simulink model "simscapePMSM"  (R2023b)
settings: Solver=VariableStepAuto  StartTime=0.0  StopTime=0.6  MaxStep=1e-4  RelTol=1e-3
undefined symbols (not defined in the file): Ld, Lq, Phif
libraries: slpidlib x2, spsDCVoltageSourceLib x1, mcbcontrolslib x1, spsPWMGenerator2LevelLib x1, eeTransforms x1, spsPermanentMagnetSynchronousMachineLib x1, spsUniversalBridgeLib x1, sps_lib x1
settings Model: Creator=HP  LastModifiedBy=HP
settings SolverCC: ZeroCrossAlgorithm=Adaptive
settings DebuggingCC: IgnoredZcDiagnostic=none

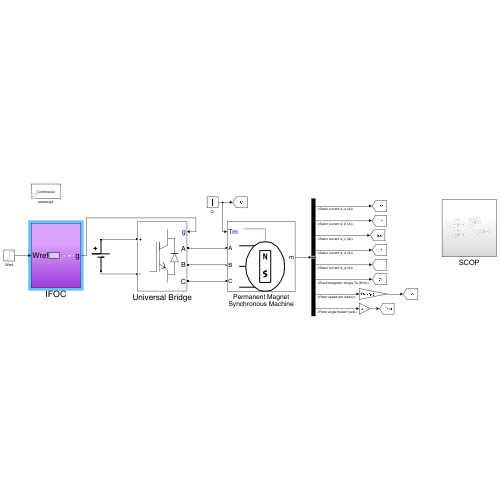
[thumbnail: Simulink's stored preview of the top-level diagram]
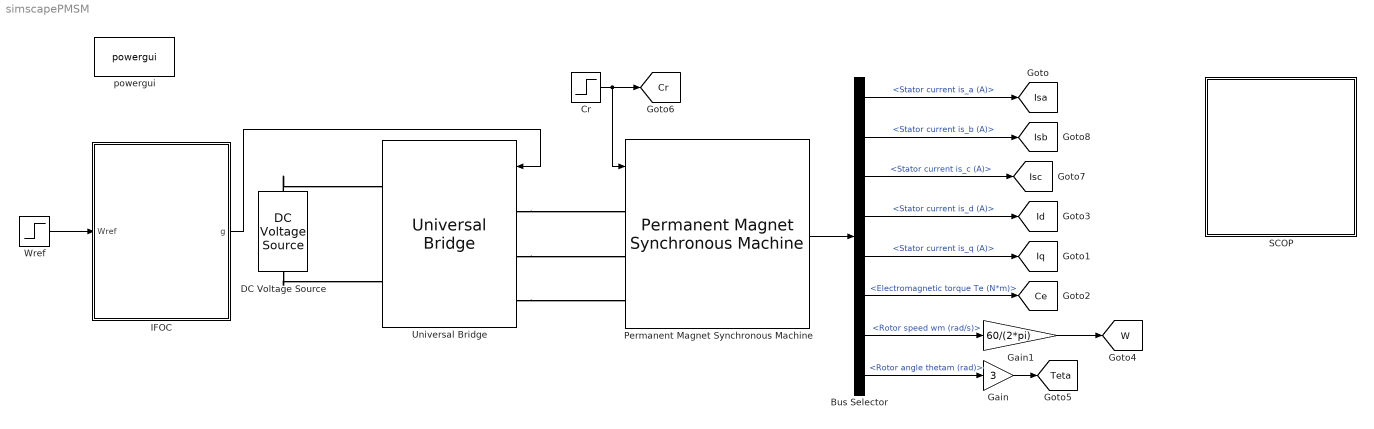
== system simscapePMSM ==
  Bus Selector : BusSelector  OutputSignals=Stator current is_a (A),Stator current is_b (A),Stator current is_c (A),Stator current is_d (A),Stator current is_q (A),Electromagnetic torque Te (N*m),Rotor speed wm (rad/s),Rotor angle thetam (rad)
  Cr : Step  Time=0.3  Before=0.5  After=10  SampleTime=0
  DC Voltage Source : spsDCVoltageSourceLib/DC Voltage Source  Amplitude=600  Measurements=None
  Gain : Gain  Gain=3
  Gain1 : Gain  Gain=60/(2*pi)
  IFOC : Subsystem
  Permanent Magnet Synchronous Machine : spsPermanentMagnetSynchronousMachineLib/Permanent Magnet Synchronous Machine  NbPhases=3  FluxDistribution=Sinusoidal  RotorType=Salient-pole  MechanicalLoad=Torque Tm  PresetModel=No  ShowDetailedParameters=on  MeasurementBus=off  Resistance=1.4  Inductance=8.5e-3  dqInductances=[0.0066,0.0038]  La=0.000395  MachineConstant=Flux linkage established by magnets (V.s)  Flux=0.1546  VoltageCst=84.124  TorqueCst=0.6957  Flat=120  Mechanical=[0.00176 0.0003881 3 0]  PolePairs=4  InitialConditions=[0,0, 0,0]  InitialConditions5ph=[0 0 0 0 0 0]  RefAngle=90 degrees behind phase A axis (modified Park)  IterativeDiscreteModel=Trapezoidal non iterative  TsBlock=-1  TsPowergui=0
  SCOP : Subsystem
  Universal Bridge : spsUniversalBridgeLib/Universal Bridge  Arms=3  SnubberResistance=1e5  SnubberCapacitance=inf  Device=IGBT / Diodes  Ron=1e-3  Lon=0  ForwardVoltages="[  0  0  ]"  ForwardVoltage=0  GTOparameters=[ 10e-6 , 20e-6 ]  IGBTparameters=[ 1e-6 , 2e-6 ]  Measurements=None  Measurements_2=None  converterType=Rectifier
  Wref : Step  Time=0.3  Before=500  After=1000  SampleTime=0
  powergui : sps_lib/powergui  Priority=1  SimulationMode=Continuous  SampleTime=50e-6  frequency=60  Iterations=50  frequencyindice=0  Pbase=100e6  ErrMax=1e-4  UnitsV=kV  UnitsW=MW  buscounter=0  FunctionMessages=off  echomessages=off  EnableUseOfTLC=off  CurrentSourceSwitches=off  DisableSnubberDevices=off  DisableRonSwitches=off  DisableVfSwitches=off  DisplayEquations=off  AutomaticDiscreteSolvers=off  SolverType=Tustin/Backward Euler (TBE)  Interpol=off  ExternalGateDelay=off  methode=off  Ts=100  x0status=blocks  SPID=on  SwTol=0  HookPort=off  NonlinearTolerance=1e-4  nMaxIteration=100  ContinueOnMaxIteration=off  RestoreLinks=warning  ResistiveCurrentMeasurement=off  Frange=[0:2:500]  Ylog=off  Xlog=on  ShowGrid=off  save=off  variable=ZData  structure=0  ZoomFFT=off  StartTime=0.0  cycles=1  DisplayStyle=1  fundamental=60  FreqAxis=off  MaxFrequency=1000  frequencyindicesteady=1  RmsSteady=1  display=off
  tag scope: Ce=global, Cr=global, Id=global, Iq=global, Isa=global, Isb=global, Isc=global, Teta=global, W=global
  wires:
  Permanent Magnet Synchronous Machine/1 -> Bus Selector/1
  Bus Selector/1 -> [Isa]  "<Stator current is_a (A)>"
  Bus Selector/4 -> [Id]  "<Stator current is_d (A)>"
  Bus Selector/5 -> [Iq]  "<Stator current is_q (A)>"
  Bus Selector/6 -> [Ce]  "<Electromagnetic torque Te (N*m)>"
  Wref/1 -> IFOC/1(Wref)
  IFOC/1(g) -> Universal Bridge/1
  Bus Selector/8 -> Gain/1  "<Rotor angle thetam (rad)>"
  Gain/1 -> [Teta]
  Cr/1 -> Permanent Magnet Synchronous Machine/1, [Cr]
  Bus Selector/2 -> [Isb]  "<Stator current is_b (A)>"
  Bus Selector/3 -> [Isc]  "<Stator current is_c (A)>"
  Gain1/1 -> [W]
  Bus Selector/7 -> Gain1/1  "<Rotor speed wm (rad/s)>"
  connections:
  DC Voltage Source/RConn1 -- Universal Bridge/RConn1
  DC Voltage Source/LConn1 -- Universal Bridge/RConn2
  Universal Bridge/LConn3 -- Permanent Magnet Synchronous Machine/LConn3
  Universal Bridge/LConn2 -- Permanent Magnet Synchronous Machine/LConn2
  Universal Bridge/LConn1 -- Permanent Magnet Synchronous Machine/LConn1

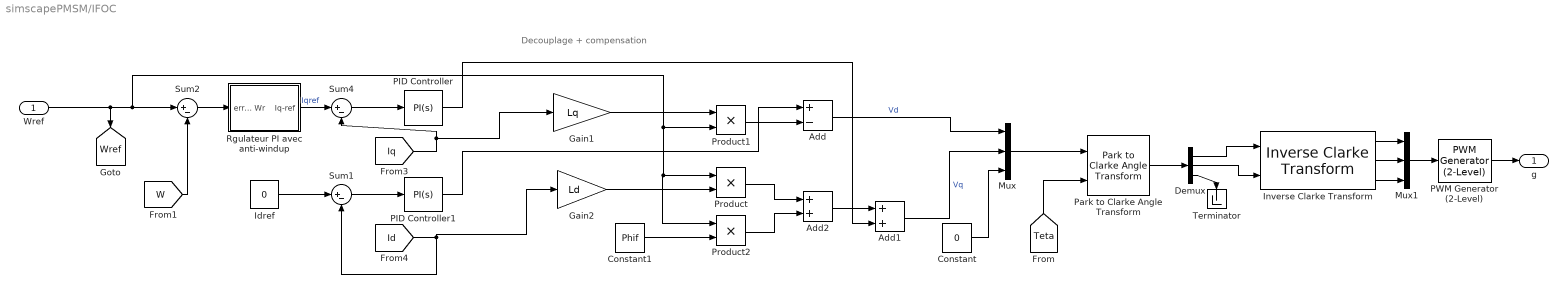
== system simscapePMSM/IFOC ==
  note: Decouplage + compensation
  Wref : Inport
  " Idref" : Constant  Value=0
  Add : Sum  Inputs=+-
  Add1 : Sum
  Add2 : Sum
  Constant : Constant  Value=0
  Constant1 : Constant  Value=Phif
  Demux : Demux  Outputs=3
  Gain1 : Gain  Gain=Lq
  Gain2 : Gain  Gain=Ld
  Inverse Clarke Transform : mcbcontrolslib/Inverse Clarke Transform  PhaseInput=Two inputs  EnPowerInv=off
      settings: LibrarySourceBlock=mcbhdllib/Controls/Math Transforms/Inverse Clarke Transform
  Mux : Mux  Inputs=3
  Mux1 : Mux  Inputs=3
  PID Controller : slpidlib/PID Controller  Controller=PI  Form=Parallel  TimeDomain=Continuous-time  UseExternalTs=off  SampleTime=-1  IntegratorMethod=Forward Euler  FilterMethod=Forward Euler  ControllerParametersSource=internal  P=100  I=20  UseKiTs=off  D=0  N=100  UseFilter=on  TunerSelectOption=Transfer Function Based (PID Tuner App)  InitialConditionSource=internal  InitialConditionForIntegrator=0  InitialConditionForFilter=0  DifferentiatorICPrevScaledInput=0  ExternalReset=none  TrackingMode=off  Kt=1  LimitOutput=off  SatLimitsSource=internal  UpperSaturationLimit=inf  LowerSaturationLimit=-inf  LinearizeAsGain=on  AntiWindupMode=none  Kb=1  LimitIntegrator=off  UpperIntegratorSaturationLimit=inf  LowerIntegratorSaturationLimit=-inf  POutMin=[]  POutMax=[]  IOutMin=[]  IOutMax=[]  DOutMin=[]  DOutMax=[]  NOutMin=[]  NOutMax=[]  SumOutMin=[]  SumOutMax=[]  SaturationOutMin=[]  SaturationOutMax=[]  PParamMin=[]  PParamMax=[]  IParamMin=[]  IParamMax=[]  DParamMin=[]  DParamMax=[]  NParamMin=[]  NParamMax=[]  KbParamMin=[]  KbParamMax=[]  KtParamMin=[]  KtParamMax=[]  KbOutMin=[]  KbOutMax=[]  KtOutMin=[]  KtOutMax=[]  IntegratorOutMin=[]  IntegratorOutMax=[]  FilterOutMin=[]  FilterOutMax=[]  SumI1OutMin=[]  SumI1OutMax=[]  SumI2OutMin=[]  SumI2OutMax=[]  SumI3OutMin=[]  SumI3OutMax=[]  SumI4OutMin=[]  SumI4OutMax=[]  SumDOutMin=[]  SumDOutMax=[]  DifferentiatorOutMin=[]  DifferentiatorOutMax=[]  FilterDiffOutCoefMin=[]  FilterDiffOutCoefMax=[]  ReciprocalOutMin=[]  ReciprocalOutMax=[]  SumDenOutMin=[]  SumDenOutMax=[]  SumNumOutMin=[]  SumNumOutMax=[]  DivideOutMin=[]  DivideOutMax=[]  UdiffTsProdOutMin=[]  UdiffTsProdOutMax=[]  NTsProdOutMin=[]  NTsProdOutMax=[]  UintegralTsProdOutMin=[]  UintegralTsProdOutMax=[]  UngainTsProdOutMin=[]  UngainTsProdOutMax=[]  ClampingZeroOutDataTypeStr=Inherit: Inherit via back propagation  ClampingZeroOutMin=[]  ClampingZeroOutMax=[]  FilterDenConstantOutDataTypeStr=Inherit: Inherit via back propagation  FilterDenConstantOutMin=[]  FilterDenConstantOutMax=[]  PCopyOutDataTypeStr=Inherit: Inherit via back propagation  PCopyOutMin=[]  PCopyOutMax=[]  NCopyOutDataTypeStr=Inherit: Inherit via back propagation  NCopyOutMin=[]  NCopyOutMax=[]  IntegratorContinuousStateAttributes=''  IntegratorStateMustResolveToSignalObject=off  IntegratorRTWStateStorageClass=Auto  FilterContinuousStateAttributes=''  FilterStateMustResolveToSignalObject=off  FilterRTWStateStorageClass=Auto  ParallelPVariant=InternalParameters  IdealPVariant=Disabled  IVariant=InternalParameters  DVariant=Disabled  IntegratorVariant=Continuous  SatVariant=Disabled  AWVariant=Passthrough  PCopyVariant=Disabled  TRVariant=Disabled  FdbkBlocksVariant=Forward  IdealPFdbkVariant=Disabled  SatFdbkVariant=Disabled  DerivativeFilterVariant=Disabled  NVariant=Disabled  NCopyVariant=Disabled_SignalSpec  FilterICVariant=Disabled  IntegratorICVariant=InternalICs  ExternalResetVariant=Disabled  TRSumVariant=Passthrough  SumFdbkVariant=Disabled  SumVariant=Sum_PI  TsampFilterVariant=InternalTs  TsampNgainVariant=Passthrough  TsampIntegralVariant=Disabled_SignalSpec  ExternalSaturationOutDataTypeStr=Inherit: Same as second input
  PID Controller1 : slpidlib/PID Controller  Controller=PI  Form=Parallel  TimeDomain=Continuous-time  UseExternalTs=off  SampleTime=-1  IntegratorMethod=Forward Euler  FilterMethod=Forward Euler  ControllerParametersSource=internal  P=100  I=20  UseKiTs=off  D=0  N=100  UseFilter=on  TunerSelectOption=Transfer Function Based (PID Tuner App)  InitialConditionSource=internal  InitialConditionForIntegrator=0  InitialConditionForFilter=0  DifferentiatorICPrevScaledInput=0  ExternalReset=none  TrackingMode=off  Kt=1  LimitOutput=off  SatLimitsSource=internal  UpperSaturationLimit=inf  LowerSaturationLimit=-inf  LinearizeAsGain=on  AntiWindupMode=none  Kb=1  LimitIntegrator=off  UpperIntegratorSaturationLimit=inf  LowerIntegratorSaturationLimit=-inf  POutMin=[]  POutMax=[]  IOutMin=[]  IOutMax=[]  DOutMin=[]  DOutMax=[]  NOutMin=[]  NOutMax=[]  SumOutMin=[]  SumOutMax=[]  SaturationOutMin=[]  SaturationOutMax=[]  PParamMin=[]  PParamMax=[]  IParamMin=[]  IParamMax=[]  DParamMin=[]  DParamMax=[]  NParamMin=[]  NParamMax=[]  KbParamMin=[]  KbParamMax=[]  KtParamMin=[]  KtParamMax=[]  KbOutMin=[]  KbOutMax=[]  KtOutMin=[]  KtOutMax=[]  IntegratorOutMin=[]  IntegratorOutMax=[]  FilterOutMin=[]  FilterOutMax=[]  SumI1OutMin=[]  SumI1OutMax=[]  SumI2OutMin=[]  SumI2OutMax=[]  SumI3OutMin=[]  SumI3OutMax=[]  SumI4OutMin=[]  SumI4OutMax=[]  SumDOutMin=[]  SumDOutMax=[]  DifferentiatorOutMin=[]  DifferentiatorOutMax=[]  FilterDiffOutCoefMin=[]  FilterDiffOutCoefMax=[]  ReciprocalOutMin=[]  ReciprocalOutMax=[]  SumDenOutMin=[]  SumDenOutMax=[]  SumNumOutMin=[]  SumNumOutMax=[]  DivideOutMin=[]  DivideOutMax=[]  UdiffTsProdOutMin=[]  UdiffTsProdOutMax=[]  NTsProdOutMin=[]  NTsProdOutMax=[]  UintegralTsProdOutMin=[]  UintegralTsProdOutMax=[]  UngainTsProdOutMin=[]  UngainTsProdOutMax=[]  ClampingZeroOutDataTypeStr=Inherit: Inherit via back propagation  ClampingZeroOutMin=[]  ClampingZeroOutMax=[]  FilterDenConstantOutDataTypeStr=Inherit: Inherit via back propagation  FilterDenConstantOutMin=[]  FilterDenConstantOutMax=[]  PCopyOutDataTypeStr=Inherit: Inherit via back propagation  PCopyOutMin=[]  PCopyOutMax=[]  NCopyOutDataTypeStr=Inherit: Inherit via back propagation  NCopyOutMin=[]  NCopyOutMax=[]  IntegratorContinuousStateAttributes=''  IntegratorStateMustResolveToSignalObject=off  IntegratorRTWStateStorageClass=Auto  FilterContinuousStateAttributes=''  FilterStateMustResolveToSignalObject=off  FilterRTWStateStorageClass=Auto  ParallelPVariant=InternalParameters  IdealPVariant=Disabled  IVariant=InternalParameters  DVariant=Disabled  IntegratorVariant=Continuous  SatVariant=Disabled  AWVariant=Passthrough  PCopyVariant=Disabled  TRVariant=Disabled  FdbkBlocksVariant=Forward  IdealPFdbkVariant=Disabled  SatFdbkVariant=Disabled  DerivativeFilterVariant=Disabled  NVariant=Disabled  NCopyVariant=Disabled_SignalSpec  FilterICVariant=Disabled  IntegratorICVariant=InternalICs  ExternalResetVariant=Disabled  TRSumVariant=Passthrough  SumFdbkVariant=Disabled  SumVariant=Sum_PI  TsampFilterVariant=InternalTs  TsampNgainVariant=Passthrough  TsampIntegralVariant=Disabled_SignalSpec  ExternalSaturationOutDataTypeStr=Inherit: Same as second input
  PWM Generator (2-Level) : spsPWMGenerator2LevelLib/PWM Generator (2-Level)  ModulatorType=Three-phase bridge (6 pulses)  ModulatorMode=Unsynchronized  Fc=27*60  Pc=90  nF=27  MinMax="[ -1  1 ]"  SamplingTechnique=Natural  ModulatingSignals=off  m=0.8  Freq=60  Phase=0  Ts=0  ShowCarrierOutport=off
  Park to Clarke Angle Transform : eeTransforms/Park to Clarke Angle Transform  AxisAlignment=Q-axis
      settings: LibrarySourceBlock=|
      | ee_sl_lib/Mathematical
      | Transforms/Park to Clarke
      | Angle Transform
  Product : Product
  Product1 : Product
  Product2 : Product
  Rgulateur PI avec anti-windup : Subsystem
  Sum1 : Sum  Inputs=|+-
  Sum2 : Sum  Inputs=|+-
  Sum4 : Sum  Inputs=|+-
  Terminator : Terminator
  g : Outport
  tag scope: Wref=global
  wires:
  Sum2/1 -> Rgulateur PI avec anti-windup/1(erreur Wr)
  Sum4/1 -> PID Controller/1
  Add/1 -> Mux/1  "Vd"
  " Idref"/1 -> Sum1/1
  Rgulateur PI avec anti-windup/1(Iq-ref) -> Sum4/1  "Iqref"
  Sum1/1 -> PID Controller1/1
  Add1/1 -> Mux/2  "Vq"
  Constant1/1 -> Product2/2
  [Id] -> Gain2/1, Sum1/2
  PID Controller/1 -> Add1/2
  Gain1/1 -> Product1/1
  Wref/1 -> [Wref], Product/1, Product2/1, Product1/2, Sum2/1
  PID Controller1/1 -> Add/1
  Gain2/1 -> Product/2
  Product2/1 -> Add2/2
  Product/1 -> Add2/1
  Product1/1 -> Add/2
  Add2/1 -> Add1/1
  [Iq] -> Gain1/1, Sum4/2
  Demux/3 -> Terminator/1
  Park to Clarke Angle Transform/1 -> Demux/1
  Mux/1 -> Park to Clarke Angle Transform/1
  Constant/1 -> Mux/3
  [W] -> Sum2/2
  [Teta] -> Park to Clarke Angle Transform/2
  Inverse Clarke Transform/1 -> Mux1/1
  Inverse Clarke Transform/2 -> Mux1/2
  Inverse Clarke Transform/3 -> Mux1/3
  Mux1/1 -> PWM Generator (2-Level)/1
  PWM Generator (2-Level)/1 -> g/1
  Demux/2 -> Inverse Clarke Transform/2
  Demux/1 -> Inverse Clarke Transform/1

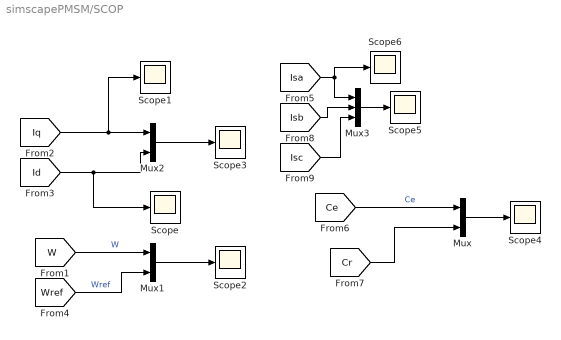
== system simscapePMSM/SCOP ==
  Mux : Mux  Inputs=2
  Mux1 : Mux  Inputs=2
  Mux2 : Mux  Inputs=2
  Mux3 : Mux  Inputs=3
  Scope{,1..6} (7 alike) : Scope
  wires:
  [Iq] -> Scope1/1, Mux2/1
  Mux2/1 -> Scope3/1
  [Id] -> Scope/1, Mux2/2
  Mux1/1 -> Scope2/1
  [W] -> Mux1/1  "W"
  [Wref] -> Mux1/2  "Wref"
  [Ce] -> Mux/1  "Ce"
  Mux/1 -> Scope4/1
  [Cr] -> Mux/2
  [Isa] -> Mux3/1, Scope6/1
  [Isb] -> Mux3/2
  [Isc] -> Mux3/3
  Mux3/1 -> Scope5/1

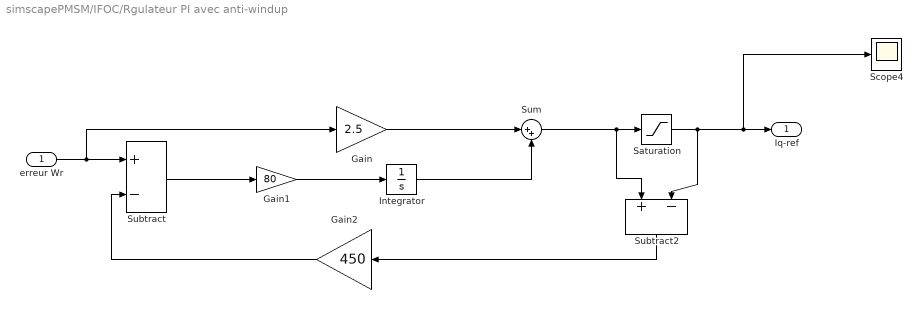
== system simscapePMSM/IFOC/Rgulateur PI avec anti-windup ==
  erreur Wr : Inport
  Gain : Gain  Gain=2.5
  Gain1 : Gain  Gain=80
  Gain2 : Gain  Gain=450
  Integrator : Integrator
  Saturation : Saturate  UpperLimit=30  LowerLimit=-30
  Scope4 : Scope
  Subtract : Sum  Inputs=+-
  Subtract2 : Sum  Inputs=+-
  Sum : Sum  Inputs=|++
  Iq-ref : Outport
  wires:
  Gain1/1 -> Integrator/1
  Gain2/1 -> Subtract/2
  Saturation/1 -> Scope4/1, Iq-ref/1, Subtract2/2
  Sum/1 -> Subtract2/1, Saturation/1
  Gain/1 -> Sum/1
  erreur Wr/1 -> Gain/1, Subtract/1
  Subtract2/1 -> Gain2/1
  Subtract/1 -> Gain1/1
  Integrator/1 -> Sum/2
